simulink model "if_mode"  (R2022b)
settings: Solver=FixedStepAuto  StartTime=0.0  StopTime=10  FixedStep=1e-4  RelTol=1e-3
values from neighbouring files (symbols this model uses):
  CurrKi = 35.0    [if_mode.sldd]
  CurrKp = 0.17    [if_mode.sldd]
  flux = 0.016884    [if_mode.sldd]
  Pn = 4.0    [if_mode.sldd]
undefined symbols (not defined in the file or in its folder): curr_d_ki, curr_d_kp, curr_q_ki, curr_q_kp, DiscIntNeverNeededParam
libraries: slpidlib x4, mcbplantlib x1, autolibpmsmexterior x1
settings Model: DataDictionary=if_mode.sldd  Creator=SSC  LastModifiedBy=SSC
settings OptimizationCC: DefaultParameterBehavior=Inlined  UseDivisionForNetSlopeComputation=on  GainParamInheritBuiltInType=on  UseFloatMulNetSlope=on  InlineInvariantSignals=on  PassReuseOutputArgsAs=Individual arguments  ZeroExternalMemoryAtStartup=off  ZeroInternalMemoryAtStartup=off  NoFixptDivByZeroProtection=on  EfficientFloat2IntCast=on  LifeSpan=1  OptimizeBlockOrder=speed  DifferentSizesBufferReuse=on  EfficientTunableParamExpr=on
settings DebuggingCC: ParameterOverflowMsg=none  ParameterUnderflowMsg=error  ParameterTunabilityLossMsg=error
settings HardwareCC: ProdBitPerPointer=32  ProdBitPerSizeT=32  ProdBitPerPtrDiffT=32  ProdLargestAtomicInteger=Long  ProdLargestAtomicFloat=Double  ProdWordSize=32  ProdLongLongMode=on  ProdHWDeviceType=ARM Compatible->ARM Cortex-M
settings SFSimCC: MATLABDynamicMemAlloc=off
settings RTWCC: Description=Embedded Coder  SystemTargetFile=ert.tlc  TemplateMakefile=ert_default_tmf  GenerateReport=on  LaunchReport=on
settings CodeAppCC: ForceParamTrailComments=on  IgnoreCustomStorageClasses=off  OperatorAnnotations=on  SimulinkDataObjDesc=on  SFDataObjDesc=on  CustomSymbolStrGlobalVar=rt$N$M  CustomSymbolStrType=$N$M  CustomSymbolStrFcn=$N$M$F  CustomSymbolStrMacro=$N$M  InsertBlockDesc=on
settings ERTTargetCC: TargetLangStandard=C99 (ISO)  CodeReplacementLibrary=ARM Cortex-M  GenerateSampleERTMain=on  IncludeMdlTerminateFcn=off  CombineSignalStateStructs=on  SupportAbsoluteTime=off  SupportComplex=off  SupportNonInlinedSFcns=on  InlinedParameterPlacement=NonHierarchical  ERTCustomFileTemplate=example_file_process.tlc  ERTFilePackagingFormat=CompactWithDataFile

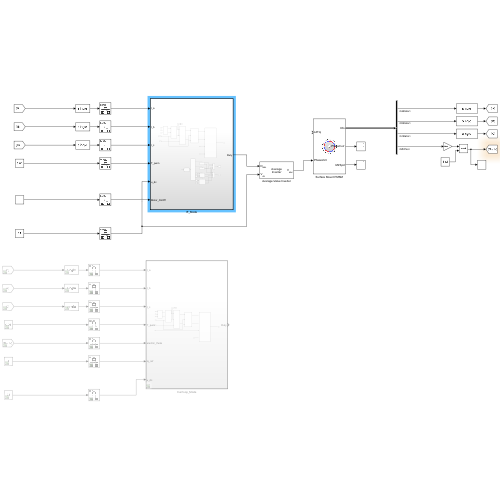
[thumbnail: Simulink's stored preview of the top-level diagram]
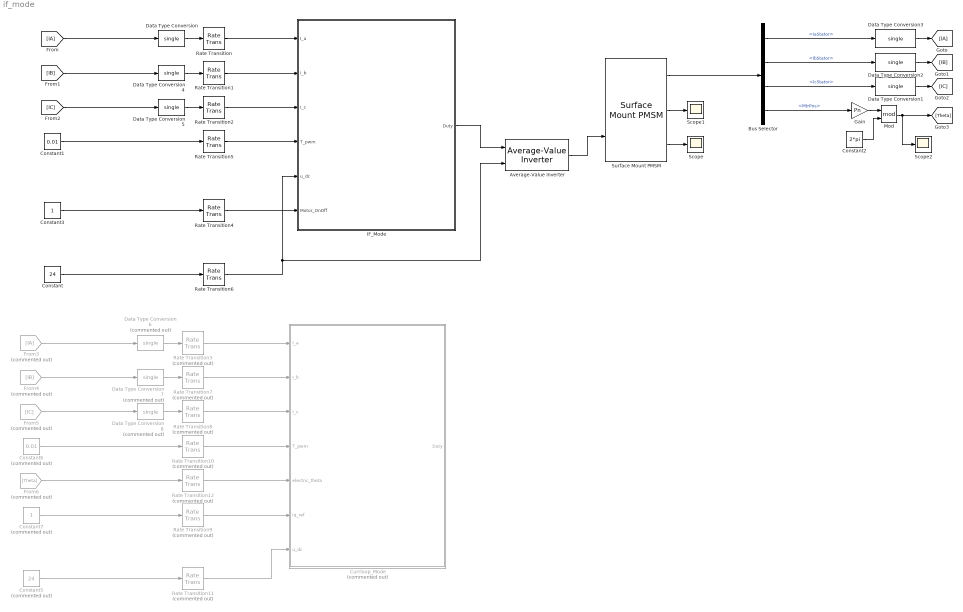
== system if_mode ==
  Average-Value Inverter : mcbplantlib/Average-Value Inverter
      settings: LibrarySourceBlock=mcblib/Electrical Systems/Inverters/Average-Value Inverter
  Bus Selector : BusSelector  OutputSignals=IaStator,IbStator,IcStator,MtrPos
  Constant : Constant  Value=24  OutDataTypeStr=single
  Constant1 : Constant  Value=0.01  OutDataTypeStr=single
  Constant2 : Constant  Value=2*pi  OutDataTypeStr=single
  Constant3 : Constant  OutDataTypeStr=single
  Constant5 : Constant  Commented=on  Value=24  OutDataTypeStr=single
  Constant6 : Constant  Commented=on  Value=0.01  OutDataTypeStr=single
  Constant7 : Constant  Commented=on  OutDataTypeStr=single
  Currloop_Mode : Subsystem  Commented=on  TreatAsAtomicUnit=on
  Data Type Conversion{,1..5} (6 alike) : DataTypeConversion  OutDataTypeStr=single  SaturateOnIntegerOverflow=off  RndMeth=Floor
  Data Type Conversion6 : DataTypeConversion  Commented=on  OutDataTypeStr=single  SaturateOnIntegerOverflow=off  RndMeth=Floor
  Data Type Conversion7 : DataTypeConversion  Commented=on  OutDataTypeStr=single  SaturateOnIntegerOverflow=off  RndMeth=Floor
  Data Type Conversion8 : DataTypeConversion  Commented=on  OutDataTypeStr=single  SaturateOnIntegerOverflow=off  RndMeth=Floor
  From3 : From  Commented=on  GotoTag=IA
  From4 : From  Commented=on  GotoTag=IB
  From5 : From  Commented=on  GotoTag=IC
  From6 : From  Commented=on  GotoTag=Theta
  Gain : Gain  Gain=Pn  OutDataTypeStr=single
  IF_Mode : Subsystem  TreatAsAtomicUnit=on
  Mod : Math  Operator=mod
  Rate Transition{,1..2,4..6} (6 alike) : RateTransition
  Rate Transition{3,7..12} (7 alike) : RateTransition  Commented=on
  Scope : Scope
  Scope1 : Scope
  Scope2 : Scope
  Surface Mount PMSM : autolibpmsmexterior/Surface Mount PMSM  port_config=Torque  sim_type=Discrete  Ts=1e-4  P=Pn  Rs=Rs  Ldq_=L  KConstText=Permanent flux linkage constant (lambda_pm):  lambda_pm=flux  Ke=223  Kt=1.323  mechanical=[75e-6,8e-5,0]  idq0=[0 0]  theta_init=0  omega_init=0  KConst=flux  lambda_pm_calc=flux  RefBlkName='autolibpmsmexterior/Surface Mount PMSM'  aMode=5  Ldq="[0.0017      0.0017]"
  wires:
  Constant/1 -> Rate Transition6/1
  Average-Value Inverter/1 -> Surface Mount PMSM/2
  Surface Mount PMSM/1 -> Bus Selector/1
  Bus Selector/1 -> Data Type Conversion3/1  "<IaStator>"
  Bus Selector/2 -> Data Type Conversion2/1  "<IbStator>"
  Bus Selector/3 -> Data Type Conversion1/1  "<IcStator>"
  Bus Selector/4 -> Gain/1  "<MtrPos>"
  Gain/1 -> Mod/1
  Mod/1 -> Scope2/1, [Theta]
  Data Type Conversion1/1 -> [IC]
  Data Type Conversion2/1 -> [IB]
  Data Type Conversion3/1 -> [IA]
  Surface Mount PMSM/3 -> Scope/1
  Surface Mount PMSM/2 -> Scope1/1
  Constant2/1 -> Mod/2
  Rate Transition2/1 -> IF_Mode/3(I_c)
  Rate Transition1/1 -> IF_Mode/2(I_b)
  Data Type Conversion/1 -> Rate Transition/1
  Data Type Conversion4/1 -> Rate Transition1/1
  [IA] -> Data Type Conversion/1
  Data Type Conversion5/1 -> Rate Transition2/1
  [IC] -> Data Type Conversion5/1
  [IB] -> Data Type Conversion4/1
  Rate Transition/1 -> IF_Mode/1(I_a)
  Rate Transition6/1 -> Average-Value Inverter/2, IF_Mode/5(u_dc)
  Constant1/1 -> Rate Transition5/1
  Rate Transition5/1 -> IF_Mode/4(T_pwm)
  Constant3/1 -> Rate Transition4/1
  Rate Transition4/1 -> IF_Mode/6(Motor_OnOff)
  Rate Transition3/1 -> Currloop_Mode/1(I_a)
  From4/1 -> Data Type Conversion7/1
  Data Type Conversion6/1 -> Rate Transition3/1
  From3/1 -> Data Type Conversion6/1
  From5/1 -> Data Type Conversion8/1
  Rate Transition11/1 -> Currloop_Mode/7(u_dc)
  Constant6/1 -> Rate Transition10/1
  Rate Transition8/1 -> Currloop_Mode/3(I_c)
  Constant5/1 -> Rate Transition11/1
  Data Type Conversion8/1 -> Rate Transition8/1
  Rate Transition7/1 -> Currloop_Mode/2(I_b)
  Constant7/1 -> Rate Transition9/1
  Data Type Conversion7/1 -> Rate Transition7/1
  Rate Transition9/1 -> Currloop_Mode/6(iq_ref)
  Rate Transition12/1 -> Currloop_Mode/5(electric_theta)
  From6/1 -> Rate Transition12/1
  Rate Transition10/1 -> Currloop_Mode/4(T_pwm)
  IF_Mode/1(Duty) -> Average-Value Inverter/1

== system if_mode/Currloop_Mode ==
  I_a : Inport
  I_b : Inport  Port=2
  I_c : Inport  Port=3
  T_pwm : Inport  Port=4
  electric_theta : Inport  Port=5
  iq_ref : Inport  Port=6
  u_dc : Inport  Port=7
  AntiPark : Subsystem
  Clark : Subsystem
  Curr_PI_Controller : Subsystem
  Park : Subsystem
  SVPWM : Subsystem
  Scope1 : Scope  NumInputPorts=2
  Duty : Outport
  wires:
  Clark/2(I_beta) -> Park/2(i_beta)  "i_beta"
  AntiPark/2(u_beta) -> SVPWM/2(U_beta)
  Park/2(i_q) -> Scope1/2, Curr_PI_Controller/2(iq_fdbk)  "i_q"
  I_c/1 -> Clark/3(I_c)
  Clark/1(I_alpha) -> Park/1(i_alpha)  "i_alpha"
  electric_theta/1 -> AntiPark/3(electric_theta), Park/3(electric_theta)
  Park/1(i_d) -> Scope1/1, Curr_PI_Controller/1(id_fdbk)  "i_d"
  Curr_PI_Controller/1(ud_ref) -> AntiPark/1(u_d)
  AntiPark/1(u_alpha) -> SVPWM/1(U_alpha)
  Curr_PI_Controller/2(uq_ref) -> AntiPark/2(u_q)
  I_a/1 -> Clark/1(I_a)
  SVPWM/1(Duty) -> Duty/1
  u_dc/1 -> SVPWM/4(u_dc)
  T_pwm/1 -> SVPWM/3(T_pwm)
  I_b/1 -> Clark/2(I_b)
  iq_ref/1 -> Curr_PI_Controller/3(iq_ref)

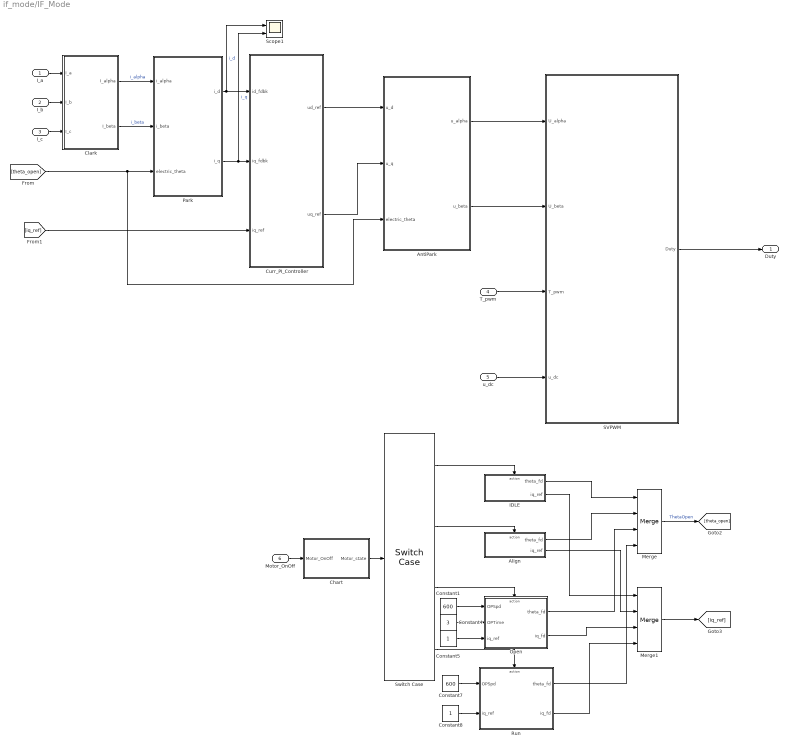
== system if_mode/IF_Mode ==
  I_a : Inport
  I_b : Inport  Port=2
  I_c : Inport  Port=3
  T_pwm : Inport  Port=4
  u_dc : Inport  Port=5
  Motor_OnOff : Inport  Port=6
  Align : Subsystem  TreatAsAtomicUnit=on
  AntiPark : Subsystem
  Chart : Stateflow chart  TreatAsAtomicUnit=on
  Clark : Subsystem
  Constant1 : Constant  Value=600  OutDataTypeStr=single
  Constant4 : Constant  Value=3  OutDataTypeStr=single
  Constant5 : Constant  OutDataTypeStr=single
  Constant7 : Constant  Value=600  OutDataTypeStr=single
  Constant8 : Constant  OutDataTypeStr=single
  Curr_PI_Controller : Subsystem
  IDLE : Subsystem  TreatAsAtomicUnit=on
  Merge : Merge  Inputs=4
  Merge1 : Merge  Inputs=4
  Open : Subsystem  TreatAsAtomicUnit=on
  Park : Subsystem
  Run : Subsystem  TreatAsAtomicUnit=on
  SVPWM : Subsystem
  Scope1 : Scope  NumInputPorts=2
  Switch Case : SwitchCase  CaseConditions={1,2,3,4}  ShowDefaultCase=off
  Duty : Outport
  wires:
  Clark/2(I_beta) -> Park/2(i_beta)  "i_beta"
  AntiPark/2(u_beta) -> SVPWM/2(U_beta)
  Park/2(i_q) -> Scope1/2, Curr_PI_Controller/2(iq_fdbk)  "i_q"
  I_c/1 -> Clark/3(I_c)
  Clark/1(I_alpha) -> Park/1(i_alpha)  "i_alpha"
  [theta_open] -> AntiPark/3(electric_theta), Park/3(electric_theta)
  Park/1(i_d) -> Scope1/1, Curr_PI_Controller/1(id_fdbk)  "i_d"
  Curr_PI_Controller/1(ud_ref) -> AntiPark/1(u_d)
  AntiPark/1(u_alpha) -> SVPWM/1(U_alpha)
  Curr_PI_Controller/2(uq_ref) -> AntiPark/2(u_q)
  I_a/1 -> Clark/1(I_a)
  SVPWM/1(Duty) -> Duty/1
  u_dc/1 -> SVPWM/4(u_dc)
  T_pwm/1 -> SVPWM/3(T_pwm)
  I_b/1 -> Clark/2(I_b)
  [iq_ref] -> Curr_PI_Controller/3(iq_ref)
  Switch Case/1 -> IDLE/Action
  Motor_OnOff/1 -> Chart/1(Motor_OnOff)
  Constant5/1 -> Open/3(iq_ref)
  Switch Case/2 -> Align/Action
  Constant4/1 -> Open/2(OPTime)
  Merge/1 -> [theta_open]  "ThetaOpen"
  Constant8/1 -> Run/2(iq_ref)
  Constant1/1 -> Open/1(OPSpd)
  Merge1/1 -> [iq_ref]
  Chart/1(Motor_state) -> Switch Case/1
  Constant7/1 -> Run/1(OPSpd)
  Switch Case/4 -> Run/Action
  Switch Case/3 -> Open/Action
  IDLE/1(theta_fd) -> Merge/1
  Align/1(theta_fd) -> Merge/2
  Open/1(theta_fd) -> Merge/3
  Run/1(theta_fd) -> Merge/4
  Run/2(iq_fd) -> Merge1/4
  Open/2(iq_fd) -> Merge1/3
  Align/2(iq_ref) -> Merge1/2
  IDLE/2(iq_ref) -> Merge1/1

== system if_mode/Currloop_Mode/AntiPark ==
  u_d : Inport
  u_q : Inport  Port=2
  electric_theta : Inport  Port=3
  Add : Sum  Inputs=+-
  Add1 : Sum
  Product{,1..3} (4 alike) : Product
  Scope : Scope  NumInputPorts=2
  Trigonometric Function : Trigonometry
  Trigonometric Function1 : Trigonometry  Operator=cos
  u_alpha : Outport
  u_beta : Outport  Port=2
  wires:
  electric_theta/1 -> Trigonometric Function1/1, Trigonometric Function/1
  u_d/1 -> Product2/1, Product/1
  Trigonometric Function1/1 -> Product/2, Product1/2
  u_q/1 -> Product1/1, Product3/1
  Trigonometric Function/1 -> Product2/2, Product3/2
  Product/1 -> Add/1
  Product3/1 -> Add/2
  Add/1 -> Scope/1, u_alpha/1
  Product2/1 -> Add1/1
  Product1/1 -> Add1/2
  Add1/1 -> Scope/2, u_beta/1

== system if_mode/Currloop_Mode/Clark ==
  I_a : Inport
  I_b : Inport  Port=2
  I_c : Inport  Port=3
  Add : Sum
  Add1 : Sum  Inputs=+-
  Add2 : Sum  Inputs=+-
  Gain : Gain  Gain=2/3
  Gain1 : Gain  Gain=1/3
  Gain2 : Gain  Gain=sqrt(3)/3
  I_alpha : Outport
  I_beta : Outport  Port=2
  wires:
  I_a/1 -> Gain/1
  I_b/1 -> Add1/1, Add/1
  I_c/1 -> Add/2, Add1/2
  Add/1 -> Gain1/1
  Add1/1 -> Gain2/1
  Gain/1 -> Add2/1
  Gain1/1 -> Add2/2
  Add2/1 -> I_alpha/1
  Gain2/1 -> I_beta/1

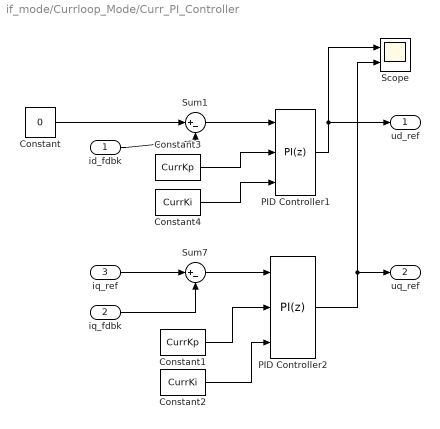
== system if_mode/Currloop_Mode/Curr_PI_Controller ==
  id_fdbk : Inport  OutDataTypeStr=single
  iq_fdbk : Inport  Port=2  OutDataTypeStr=single
  iq_ref : Inport  Port=3  OutDataTypeStr=single
  Constant : Constant  Value=0  OutDataTypeStr=single
  Constant1 : Constant  Value=CurrKp  OutDataTypeStr=single
  Constant2 : Constant  Value=CurrKi  OutDataTypeStr=single
  Constant3 : Constant  Value=CurrKp  OutDataTypeStr=single
  Constant4 : Constant  Value=CurrKi  OutDataTypeStr=single
  PID Controller1 : slpidlib/PID Controller  Controller=PI  Form=Parallel  TimeDomain=Discrete-time  UseExternalTs=off  SampleTime=-1  IntegratorMethod=Forward Euler  FilterMethod=Forward Euler  ControllerParametersSource=external  P=curr_d_kp  I=curr_d_ki  UseKiTs=off  D=0  N=100  UseFilter=on  TunerSelectOption=Transfer Function Based (PID Tuner App)  InitialConditionSource=internal  InitialConditionForIntegrator=0  InitialConditionForFilter=0  DifferentiatorICPrevScaledInput=0  ExternalReset=none  TrackingMode=off  Kt=1  LimitOutput=on  SatLimitsSource=internal  UpperSaturationLimit=24*0.9/sqrt(3)  LowerSaturationLimit=-24*0.9/sqrt(3)  LinearizeAsGain=on  AntiWindupMode=clamping  Kb=1  LimitIntegrator=off  UpperIntegratorSaturationLimit=inf  LowerIntegratorSaturationLimit=-inf  PGainOutDataTypeStr=single  PProdOutDataTypeStr=single  POutMin=[]  POutMax=[]  IGainOutDataTypeStr=int16  IProdOutDataTypeStr=int16  IOutMin=[]  IOutMax=[]  DOutMin=[]  DOutMax=[]  NOutMin=[]  NOutMax=[]  SumOutDataTypeStr=single  SumOutMin=[]  SumOutMax=[]  SaturationOutDataTypeStr=single  SaturationOutMin=[]  SaturationOutMax=[]  PParamMin=[]  PParamMax=[]  IParamMin=[]  IParamMax=[]  DParamMin=[]  DParamMax=[]  NParamMin=[]  NParamMax=[]  KbParamMin=[]  KbParamMax=[]  KtParamMin=[]  KtParamMax=[]  KbOutMin=[]  KbOutMax=[]  KtOutMin=[]  KtOutMax=[]  IntegratorOutMin=[]  IntegratorOutMax=[]  FilterOutMin=[]  FilterOutMax=[]  SumI1OutMin=[]  SumI1OutMax=[]  SumI2OutMin=[]  SumI2OutMax=[]  SumI3OutMin=[]  SumI3OutMax=[]  SumI4OutMin=[]  SumI4OutMax=[]  SumDOutMin=[]  SumDOutMax=[]  DifferentiatorOutMin=[]  DifferentiatorOutMax=[]  FilterDiffOutCoefMin=[]  FilterDiffOutCoefMax=[]  ReciprocalOutMin=[]  ReciprocalOutMax=[]  SumDenOutMin=[]  SumDenOutMax=[]  SumNumOutMin=[]  SumNumOutMax=[]  DivideOutMin=[]  DivideOutMax=[]  UdiffTsProdOutMin=[]  UdiffTsProdOutMax=[]  NTsProdOutMin=[]  NTsProdOutMax=[]  UintegralTsProdOutMin=[]  UintegralTsProdOutMax=[]  UngainTsProdOutMin=[]  UngainTsProdOutMax=[]  ClampingZeroOutDataTypeStr=Inherit: Inherit via back propagation  ClampingZeroOutMin=[]  ClampingZeroOutMax=[]  FilterDenConstantOutDataTypeStr=Inherit: Inherit via back propagation  FilterDenConstantOutMin=[]  FilterDenConstantOutMax=[]  PCopyOutDataTypeStr=Inherit: Inherit via back propagation  PCopyOutMin=[]  PCopyOutMax=[]  NCopyOutDataTypeStr=Inherit: Inherit via back propagation  NCopyOutMin=[]  NCopyOutMax=[]  IntegratorContinuousStateAttributes=''  IntegratorStateMustResolveToSignalObject=off  IntegratorRTWStateStorageClass=Auto  FilterContinuousStateAttributes=''  FilterStateMustResolveToSignalObject=off  FilterRTWStateStorageClass=Auto  ParallelPVariant=ExternalParameters  IdealPVariant=Disabled  IVariant=ExternalParameters  DVariant=Disabled  IntegratorVariant=Discrete  SatVariant=Enabled  AWVariant=DiscClampingParallel  PCopyVariant=Disabled  TRVariant=Disabled  FdbkBlocksVariant=Forward  IdealPFdbkVariant=Disabled  SatFdbkVariant=Disabled  DerivativeFilterVariant=Disabled  NVariant=Disabled  NCopyVariant=Disabled_SignalSpec  FilterICVariant=Disabled  IntegratorICVariant=InternalICs  ExternalResetVariant=Disabled  TRSumVariant=Passthrough  SumFdbkVariant=Disabled  SumVariant=Sum_PI  TsampFilterVariant=InternalTs  TsampNgainVariant=Passthrough  TsampIntegralVariant=Passthrough  ExternalSaturationOutDataTypeStr=Inherit: Same as second input
  PID Controller2 : slpidlib/PID Controller  Controller=PI  Form=Parallel  TimeDomain=Discrete-time  UseExternalTs=off  SampleTime=-1  IntegratorMethod=Forward Euler  FilterMethod=Forward Euler  ControllerParametersSource=external  P=curr_q_kp  I=curr_q_ki  UseKiTs=off  D=0  N=100  UseFilter=on  TunerSelectOption=Transfer Function Based (PID Tuner App)  InitialConditionSource=internal  InitialConditionForIntegrator=0  InitialConditionForFilter=0  DifferentiatorICPrevScaledInput=0  ExternalReset=none  TrackingMode=off  Kt=1  LimitOutput=on  SatLimitsSource=internal  UpperSaturationLimit=24*0.9/sqrt(3)  LowerSaturationLimit=-24*0.9/sqrt(3)  LinearizeAsGain=on  AntiWindupMode=clamping  Kb=1  LimitIntegrator=off  UpperIntegratorSaturationLimit=inf  LowerIntegratorSaturationLimit=-inf  PGainOutDataTypeStr=single  PProdOutDataTypeStr=single  POutMin=[]  POutMax=[]  IGainOutDataTypeStr=single  IProdOutDataTypeStr=single  IOutMin=[]  IOutMax=[]  DOutMin=[]  DOutMax=[]  NOutMin=[]  NOutMax=[]  SumOutDataTypeStr=single  SumOutMin=[]  SumOutMax=[]  SaturationOutDataTypeStr=single  SaturationOutMin=[]  SaturationOutMax=[]  PParamMin=[]  PParamMax=[]  IParamMin=[]  IParamMax=[]  DParamMin=[]  DParamMax=[]  NParamMin=[]  NParamMax=[]  KbParamMin=[]  KbParamMax=[]  KtParamMin=[]  KtParamMax=[]  KbOutMin=[]  KbOutMax=[]  KtOutMin=[]  KtOutMax=[]  IntegratorOutMin=[]  IntegratorOutMax=[]  FilterOutMin=[]  FilterOutMax=[]  SumI1OutMin=[]  SumI1OutMax=[]  SumI2OutMin=[]  SumI2OutMax=[]  SumI3OutMin=[]  SumI3OutMax=[]  SumI4OutMin=[]  SumI4OutMax=[]  SumDOutMin=[]  SumDOutMax=[]  DifferentiatorOutMin=[]  DifferentiatorOutMax=[]  FilterDiffOutCoefMin=[]  FilterDiffOutCoefMax=[]  ReciprocalOutMin=[]  ReciprocalOutMax=[]  SumDenOutMin=[]  SumDenOutMax=[]  SumNumOutMin=[]  SumNumOutMax=[]  DivideOutMin=[]  DivideOutMax=[]  UdiffTsProdOutMin=[]  UdiffTsProdOutMax=[]  NTsProdOutMin=[]  NTsProdOutMax=[]  UintegralTsProdOutMin=[]  UintegralTsProdOutMax=[]  UngainTsProdOutMin=[]  UngainTsProdOutMax=[]  ClampingZeroOutDataTypeStr=Inherit: Inherit via back propagation  ClampingZeroOutMin=[]  ClampingZeroOutMax=[]  FilterDenConstantOutDataTypeStr=Inherit: Inherit via back propagation  FilterDenConstantOutMin=[]  FilterDenConstantOutMax=[]  PCopyOutDataTypeStr=Inherit: Inherit via back propagation  PCopyOutMin=[]  PCopyOutMax=[]  NCopyOutDataTypeStr=Inherit: Inherit via back propagation  NCopyOutMin=[]  NCopyOutMax=[]  IntegratorContinuousStateAttributes=''  IntegratorStateMustResolveToSignalObject=off  IntegratorRTWStateStorageClass=Auto  FilterContinuousStateAttributes=''  FilterStateMustResolveToSignalObject=off  FilterRTWStateStorageClass=Auto  ParallelPVariant=ExternalParameters  IdealPVariant=Disabled  IVariant=ExternalParameters  DVariant=Disabled  IntegratorVariant=Discrete  SatVariant=Enabled  AWVariant=DiscClampingParallel  PCopyVariant=Disabled  TRVariant=Disabled  FdbkBlocksVariant=Forward  IdealPFdbkVariant=Disabled  SatFdbkVariant=Disabled  DerivativeFilterVariant=Disabled  NVariant=Disabled  NCopyVariant=Disabled_SignalSpec  FilterICVariant=Disabled  IntegratorICVariant=InternalICs  ExternalResetVariant=Disabled  TRSumVariant=Passthrough  SumFdbkVariant=Disabled  SumVariant=Sum_PI  TsampFilterVariant=InternalTs  TsampNgainVariant=Passthrough  TsampIntegralVariant=Passthrough  ExternalSaturationOutDataTypeStr=Inherit: Same as second input
  Scope : Scope  NumInputPorts=2
  Sum1 : Sum  Inputs=|+-  AccumDataTypeStr=single  OutDataTypeStr=single
  Sum7 : Sum  Inputs=|+-  AccumDataTypeStr=single  OutDataTypeStr=single
  ud_ref : Outport  OutDataTypeStr=single
  uq_ref : Outport  Port=2  OutDataTypeStr=single
  wires:
  id_fdbk/1 -> Sum1/2
  Constant/1 -> Sum1/1
  iq_fdbk/1 -> Sum7/2
  Sum1/1 -> PID Controller1/1
  PID Controller1/1 -> Scope/1, ud_ref/1
  PID Controller2/1 -> Scope/2, uq_ref/1
  iq_ref/1 -> Sum7/1
  Constant3/1 -> PID Controller1/2
  Constant4/1 -> PID Controller1/3
  Constant1/1 -> PID Controller2/2
  Constant2/1 -> PID Controller2/3
  Sum7/1 -> PID Controller2/1

== system if_mode/Currloop_Mode/Park ==
  i_alpha : Inport
  i_beta : Inport  Port=2
  electric_theta : Inport  Port=3
  Add : Sum
  Add1 : Sum  Inputs=-+
  Product{,1..3} (4 alike) : Product
  Scope : Scope  NumInputPorts=2
  Trigonometric Function : Trigonometry
  Trigonometric Function1 : Trigonometry  Operator=cos
  i_d : Outport
  i_q : Outport  Port=2
  wires:
  electric_theta/1 -> Trigonometric Function1/1, Trigonometric Function/1
  i_alpha/1 -> Product2/1, Product/1
  Trigonometric Function1/1 -> Product3/2, Product/2
  i_beta/1 -> Product3/1, Product1/1
  Trigonometric Function/1 -> Product2/2, Product1/2
  Product/1 -> Add/1
  Product1/1 -> Add/2
  Product2/1 -> Add1/1
  Product3/1 -> Add1/2
  Add/1 -> Scope/1, i_d/1
  Add1/1 -> Scope/2, i_q/1

== system if_mode/Currloop_Mode/SVPWM ==
  U_alpha : Inport
  U_beta : Inport  Port=2
  T_pwm : Inport  Port=3
  u_dc : Inport  Port=4
  Constant : Constant
  Duty_Caculator : Subsystem
  Gain : Gain  Gain=2
  Mux : Mux  Inputs=3
  Sector_Select : Subsystem
  Sum : Sum  Inputs=|-+
  T4_T6_Caculator : Subsystem
  X_Y_Z_Caculator : Subsystem
  Duty : Outport
  wires:
  U_alpha/1 -> X_Y_Z_Caculator/1(u_alpha), Sector_Select/1(u_alpha)
  U_beta/1 -> X_Y_Z_Caculator/2(u_beta), Sector_Select/2(u_beta)
  T_pwm/1 -> Duty_Caculator/4(T_pwm), T4_T6_Caculator/5(T_pwm), X_Y_Z_Caculator/3(T_pwm)
  u_dc/1 -> X_Y_Z_Caculator/4(U_dc)
  X_Y_Z_Caculator/1(X) -> T4_T6_Caculator/2(X)
  X_Y_Z_Caculator/2(Y) -> T4_T6_Caculator/3(Y)
  X_Y_Z_Caculator/3(Z) -> T4_T6_Caculator/4(Z)
  Sector_Select/1(N) -> T4_T6_Caculator/1(N), Duty_Caculator/1(N)
  T4_T6_Caculator/2(T6) -> Duty_Caculator/3(T6)
  T4_T6_Caculator/1(T4) -> Duty_Caculator/2(T4)
  Duty_Caculator/2(Dutyb) -> Mux/2
  Duty_Caculator/1(Dutya) -> Mux/1
  Duty_Caculator/3(Dutyc) -> Mux/3
  Sum/1 -> Duty/1
  Constant/1 -> Sum/2
  Mux/1 -> Gain/1
  Gain/1 -> Sum/1

== system if_mode/IF_Mode/Align ==
  Action Port : ActionPort  ActionPortLabel=case [ 2 ]:
  Constant : Constant  Value=0  OutDataTypeStr=single
  Constant1 : Constant  Value=2  OutDataTypeStr=single
  theta_fd : Outport
  iq_ref : Outport  Port=2
  wires:
  Constant1/1 -> iq_ref/1
  Constant/1 -> theta_fd/1

== system if_mode/IF_Mode/AntiPark ==
  u_d : Inport
  u_q : Inport  Port=2
  electric_theta : Inport  Port=3
  Add : Sum  Inputs=+-
  Add1 : Sum
  Product{,1..3} (4 alike) : Product
  Scope : Scope  NumInputPorts=2
  Trigonometric Function : Trigonometry
  Trigonometric Function1 : Trigonometry  Operator=cos
  u_alpha : Outport
  u_beta : Outport  Port=2
  wires:
  electric_theta/1 -> Trigonometric Function1/1, Trigonometric Function/1
  u_d/1 -> Product2/1, Product/1
  Trigonometric Function1/1 -> Product/2, Product1/2
  u_q/1 -> Product1/1, Product3/1
  Trigonometric Function/1 -> Product2/2, Product3/2
  Product/1 -> Add/1
  Product3/1 -> Add/2
  Add/1 -> Scope/1, u_alpha/1
  Product2/1 -> Add1/1
  Product1/1 -> Add1/2
  Add1/1 -> Scope/2, u_beta/1

== system if_mode/IF_Mode/Clark ==
  I_a : Inport
  I_b : Inport  Port=2
  I_c : Inport  Port=3
  Add : Sum
  Add1 : Sum  Inputs=+-
  Add2 : Sum  Inputs=+-
  Gain : Gain  Gain=2/3
  Gain1 : Gain  Gain=1/3
  Gain2 : Gain  Gain=sqrt(3)/3
  I_alpha : Outport
  I_beta : Outport  Port=2
  wires:
  I_a/1 -> Gain/1
  I_b/1 -> Add1/1, Add/1
  I_c/1 -> Add/2, Add1/2
  Add/1 -> Gain1/1
  Add1/1 -> Gain2/1
  Gain/1 -> Add2/1
  Gain1/1 -> Add2/2
  Add2/1 -> I_alpha/1
  Gain2/1 -> I_beta/1

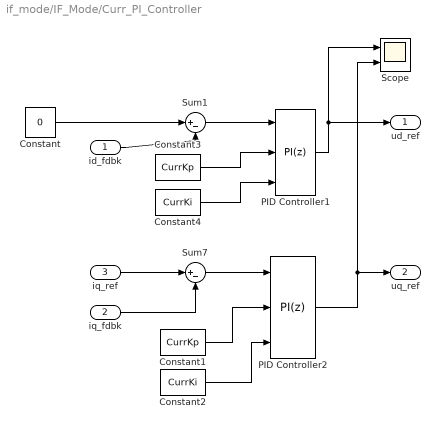
== system if_mode/IF_Mode/Curr_PI_Controller ==
  id_fdbk : Inport  OutDataTypeStr=single
  iq_fdbk : Inport  Port=2  OutDataTypeStr=single
  iq_ref : Inport  Port=3  OutDataTypeStr=single
  Constant : Constant  Value=0  OutDataTypeStr=single
  Constant1 : Constant  Value=CurrKp  OutDataTypeStr=single
  Constant2 : Constant  Value=CurrKi  OutDataTypeStr=single
  Constant3 : Constant  Value=CurrKp  OutDataTypeStr=single
  Constant4 : Constant  Value=CurrKi  OutDataTypeStr=single
  PID Controller1 : slpidlib/PID Controller  Controller=PI  Form=Parallel  TimeDomain=Discrete-time  UseExternalTs=off  SampleTime=-1  IntegratorMethod=Forward Euler  FilterMethod=Forward Euler  ControllerParametersSource=external  P=curr_d_kp  I=curr_d_ki  UseKiTs=off  D=0  N=100  UseFilter=on  TunerSelectOption=Transfer Function Based (PID Tuner App)  InitialConditionSource=internal  InitialConditionForIntegrator=0  InitialConditionForFilter=0  DifferentiatorICPrevScaledInput=0  ExternalReset=none  TrackingMode=off  Kt=1  LimitOutput=on  SatLimitsSource=internal  UpperSaturationLimit=24*0.9/sqrt(3)  LowerSaturationLimit=-24*0.9/sqrt(3)  LinearizeAsGain=on  AntiWindupMode=clamping  Kb=1  LimitIntegrator=off  UpperIntegratorSaturationLimit=inf  LowerIntegratorSaturationLimit=-inf  PGainOutDataTypeStr=single  PProdOutDataTypeStr=single  POutMin=[]  POutMax=[]  IGainOutDataTypeStr=int16  IProdOutDataTypeStr=int16  IOutMin=[]  IOutMax=[]  DOutMin=[]  DOutMax=[]  NOutMin=[]  NOutMax=[]  SumOutDataTypeStr=single  SumOutMin=[]  SumOutMax=[]  SaturationOutDataTypeStr=single  SaturationOutMin=[]  SaturationOutMax=[]  PParamMin=[]  PParamMax=[]  IParamMin=[]  IParamMax=[]  DParamMin=[]  DParamMax=[]  NParamMin=[]  NParamMax=[]  KbParamMin=[]  KbParamMax=[]  KtParamMin=[]  KtParamMax=[]  KbOutMin=[]  KbOutMax=[]  KtOutMin=[]  KtOutMax=[]  IntegratorOutMin=[]  IntegratorOutMax=[]  FilterOutMin=[]  FilterOutMax=[]  SumI1OutMin=[]  SumI1OutMax=[]  SumI2OutMin=[]  SumI2OutMax=[]  SumI3OutMin=[]  SumI3OutMax=[]  SumI4OutMin=[]  SumI4OutMax=[]  SumDOutMin=[]  SumDOutMax=[]  DifferentiatorOutMin=[]  DifferentiatorOutMax=[]  FilterDiffOutCoefMin=[]  FilterDiffOutCoefMax=[]  ReciprocalOutMin=[]  ReciprocalOutMax=[]  SumDenOutMin=[]  SumDenOutMax=[]  SumNumOutMin=[]  SumNumOutMax=[]  DivideOutMin=[]  DivideOutMax=[]  UdiffTsProdOutMin=[]  UdiffTsProdOutMax=[]  NTsProdOutMin=[]  NTsProdOutMax=[]  UintegralTsProdOutMin=[]  UintegralTsProdOutMax=[]  UngainTsProdOutMin=[]  UngainTsProdOutMax=[]  ClampingZeroOutDataTypeStr=Inherit: Inherit via back propagation  ClampingZeroOutMin=[]  ClampingZeroOutMax=[]  FilterDenConstantOutDataTypeStr=Inherit: Inherit via back propagation  FilterDenConstantOutMin=[]  FilterDenConstantOutMax=[]  PCopyOutDataTypeStr=Inherit: Inherit via back propagation  PCopyOutMin=[]  PCopyOutMax=[]  NCopyOutDataTypeStr=Inherit: Inherit via back propagation  NCopyOutMin=[]  NCopyOutMax=[]  IntegratorContinuousStateAttributes=''  IntegratorStateMustResolveToSignalObject=off  IntegratorRTWStateStorageClass=Auto  FilterContinuousStateAttributes=''  FilterStateMustResolveToSignalObject=off  FilterRTWStateStorageClass=Auto  ParallelPVariant=ExternalParameters  IdealPVariant=Disabled  IVariant=ExternalParameters  DVariant=Disabled  IntegratorVariant=Discrete  SatVariant=Enabled  AWVariant=DiscClampingParallel  PCopyVariant=Disabled  TRVariant=Disabled  FdbkBlocksVariant=Forward  IdealPFdbkVariant=Disabled  SatFdbkVariant=Disabled  DerivativeFilterVariant=Disabled  NVariant=Disabled  NCopyVariant=Disabled_SignalSpec  FilterICVariant=Disabled  IntegratorICVariant=InternalICs  ExternalResetVariant=Disabled  TRSumVariant=Passthrough  SumFdbkVariant=Disabled  SumVariant=Sum_PI  TsampFilterVariant=InternalTs  TsampNgainVariant=Passthrough  TsampIntegralVariant=Passthrough  ExternalSaturationOutDataTypeStr=Inherit: Same as second input
  PID Controller2 : slpidlib/PID Controller  Controller=PI  Form=Parallel  TimeDomain=Discrete-time  UseExternalTs=off  SampleTime=-1  IntegratorMethod=Forward Euler  FilterMethod=Forward Euler  ControllerParametersSource=external  P=curr_q_kp  I=curr_q_ki  UseKiTs=off  D=0  N=100  UseFilter=on  TunerSelectOption=Transfer Function Based (PID Tuner App)  InitialConditionSource=internal  InitialConditionForIntegrator=0  InitialConditionForFilter=0  DifferentiatorICPrevScaledInput=0  ExternalReset=none  TrackingMode=off  Kt=1  LimitOutput=on  SatLimitsSource=internal  UpperSaturationLimit=24*0.9/sqrt(3)  LowerSaturationLimit=-24*0.9/sqrt(3)  LinearizeAsGain=on  AntiWindupMode=clamping  Kb=1  LimitIntegrator=off  UpperIntegratorSaturationLimit=inf  LowerIntegratorSaturationLimit=-inf  PGainOutDataTypeStr=single  PProdOutDataTypeStr=single  POutMin=[]  POutMax=[]  IGainOutDataTypeStr=single  IProdOutDataTypeStr=single  IOutMin=[]  IOutMax=[]  DOutMin=[]  DOutMax=[]  NOutMin=[]  NOutMax=[]  SumOutDataTypeStr=single  SumOutMin=[]  SumOutMax=[]  SaturationOutDataTypeStr=single  SaturationOutMin=[]  SaturationOutMax=[]  PParamMin=[]  PParamMax=[]  IParamMin=[]  IParamMax=[]  DParamMin=[]  DParamMax=[]  NParamMin=[]  NParamMax=[]  KbParamMin=[]  KbParamMax=[]  KtParamMin=[]  KtParamMax=[]  KbOutMin=[]  KbOutMax=[]  KtOutMin=[]  KtOutMax=[]  IntegratorOutMin=[]  IntegratorOutMax=[]  FilterOutMin=[]  FilterOutMax=[]  SumI1OutMin=[]  SumI1OutMax=[]  SumI2OutMin=[]  SumI2OutMax=[]  SumI3OutMin=[]  SumI3OutMax=[]  SumI4OutMin=[]  SumI4OutMax=[]  SumDOutMin=[]  SumDOutMax=[]  DifferentiatorOutMin=[]  DifferentiatorOutMax=[]  FilterDiffOutCoefMin=[]  FilterDiffOutCoefMax=[]  ReciprocalOutMin=[]  ReciprocalOutMax=[]  SumDenOutMin=[]  SumDenOutMax=[]  SumNumOutMin=[]  SumNumOutMax=[]  DivideOutMin=[]  DivideOutMax=[]  UdiffTsProdOutMin=[]  UdiffTsProdOutMax=[]  NTsProdOutMin=[]  NTsProdOutMax=[]  UintegralTsProdOutMin=[]  UintegralTsProdOutMax=[]  UngainTsProdOutMin=[]  UngainTsProdOutMax=[]  ClampingZeroOutDataTypeStr=Inherit: Inherit via back propagation  ClampingZeroOutMin=[]  ClampingZeroOutMax=[]  FilterDenConstantOutDataTypeStr=Inherit: Inherit via back propagation  FilterDenConstantOutMin=[]  FilterDenConstantOutMax=[]  PCopyOutDataTypeStr=Inherit: Inherit via back propagation  PCopyOutMin=[]  PCopyOutMax=[]  NCopyOutDataTypeStr=Inherit: Inherit via back propagation  NCopyOutMin=[]  NCopyOutMax=[]  IntegratorContinuousStateAttributes=''  IntegratorStateMustResolveToSignalObject=off  IntegratorRTWStateStorageClass=Auto  FilterContinuousStateAttributes=''  FilterStateMustResolveToSignalObject=off  FilterRTWStateStorageClass=Auto  ParallelPVariant=ExternalParameters  IdealPVariant=Disabled  IVariant=ExternalParameters  DVariant=Disabled  IntegratorVariant=Discrete  SatVariant=Enabled  AWVariant=DiscClampingParallel  PCopyVariant=Disabled  TRVariant=Disabled  FdbkBlocksVariant=Forward  IdealPFdbkVariant=Disabled  SatFdbkVariant=Disabled  DerivativeFilterVariant=Disabled  NVariant=Disabled  NCopyVariant=Disabled_SignalSpec  FilterICVariant=Disabled  IntegratorICVariant=InternalICs  ExternalResetVariant=Disabled  TRSumVariant=Passthrough  SumFdbkVariant=Disabled  SumVariant=Sum_PI  TsampFilterVariant=InternalTs  TsampNgainVariant=Passthrough  TsampIntegralVariant=Passthrough  ExternalSaturationOutDataTypeStr=Inherit: Same as second input
  Scope : Scope  NumInputPorts=2
  Sum1 : Sum  Inputs=|+-  AccumDataTypeStr=single  OutDataTypeStr=single
  Sum7 : Sum  Inputs=|+-  AccumDataTypeStr=single  OutDataTypeStr=single
  ud_ref : Outport  OutDataTypeStr=single
  uq_ref : Outport  Port=2  OutDataTypeStr=single
  wires:
  id_fdbk/1 -> Sum1/2
  Constant/1 -> Sum1/1
  iq_fdbk/1 -> Sum7/2
  Sum1/1 -> PID Controller1/1
  PID Controller1/1 -> Scope/1, ud_ref/1
  PID Controller2/1 -> Scope/2, uq_ref/1
  iq_ref/1 -> Sum7/1
  Constant3/1 -> PID Controller1/2
  Constant4/1 -> PID Controller1/3
  Constant1/1 -> PID Controller2/2
  Constant2/1 -> PID Controller2/3
  Sum7/1 -> PID Controller2/1

== system if_mode/IF_Mode/IDLE ==
  Action Port : ActionPort  ActionPortLabel=case [ 1 ]:
  Constant : Constant  Value=0  OutDataTypeStr=single
  Constant1 : Constant  Value=0  OutDataTypeStr=single
  theta_fd : Outport
  iq_ref : Outport  Port=2
  wires:
  Constant1/1 -> iq_ref/1
  Constant/1 -> theta_fd/1

== system if_mode/IF_Mode/Open ==
  OPSpd : Inport  OutDataTypeStr=single  PortDimensions=1
  OPTime : Inport  Port=2  OutDataTypeStr=single  PortDimensions=1
  iq_ref : Inport  Port=3
  Action Port : ActionPort  ActionPortLabel=case [ 3 ]:
  Constant1 : Constant  Value=2*pi  OutDataTypeStr=single
  Constant4 : Constant  OutDataTypeStr=single
  Discrete-Time Integrator : DiscreteIntegrator  SampleTime=-1  ICPrevOutput=DiscIntNeverNeededParam  ICPrevScaledInput=DiscIntNeverNeededParam
  Discrete-Time Integrator1 : DiscreteIntegrator  SampleTime=-1  ICPrevOutput=DiscIntNeverNeededParam  ICPrevScaledInput=DiscIntNeverNeededParam
  Divide : Product  Inputs=*/  OutDataTypeStr=single
  Gain : Gain  Gain=Pn
  Gain1 : Gain  Gain=pi/30  OutDataTypeStr=single
  Mod : Math  Operator=mod
  Product : Product  OutDataTypeStr=single
  theta_fd : Outport
  iq_fd : Outport  Port=2
  wires:
  iq_ref/1 -> iq_fd/1
  Constant4/1 -> Divide/1
  Constant1/1 -> Mod/2
  Discrete-Time Integrator1/1 -> Mod/1
  Gain1/1 -> Gain/1
  Divide/1 -> Product/2
  Discrete-Time Integrator/1 -> Discrete-Time Integrator1/1
  Mod/1 -> theta_fd/1
  Gain/1 -> Product/1
  Product/1 -> Discrete-Time Integrator/1
  OPSpd/1 -> Gain1/1
  OPTime/1 -> Divide/2

== system if_mode/IF_Mode/Park ==
  i_alpha : Inport
  i_beta : Inport  Port=2
  electric_theta : Inport  Port=3
  Add : Sum
  Add1 : Sum  Inputs=-+
  Product{,1..3} (4 alike) : Product
  Scope : Scope  NumInputPorts=2
  Trigonometric Function : Trigonometry
  Trigonometric Function1 : Trigonometry  Operator=cos
  i_d : Outport
  i_q : Outport  Port=2
  wires:
  electric_theta/1 -> Trigonometric Function1/1, Trigonometric Function/1
  i_alpha/1 -> Product2/1, Product/1
  Trigonometric Function1/1 -> Product3/2, Product/2
  i_beta/1 -> Product3/1, Product1/1
  Trigonometric Function/1 -> Product2/2, Product1/2
  Product/1 -> Add/1
  Product1/1 -> Add/2
  Product2/1 -> Add1/1
  Product3/1 -> Add1/2
  Add/1 -> Scope/1, i_d/1
  Add1/1 -> Scope/2, i_q/1

== system if_mode/IF_Mode/Run ==
  OPSpd : Inport  OutDataTypeStr=single  PortDimensions=1
  iq_ref : Inport  Port=2
  Action Port : ActionPort  ActionPortLabel=case [ 4 ]:
  Constant1 : Constant  Value=2*pi  OutDataTypeStr=single
  Discrete-Time Integrator1 : DiscreteIntegrator  SampleTime=-1  ICPrevOutput=DiscIntNeverNeededParam  ICPrevScaledInput=DiscIntNeverNeededParam
  Gain : Gain  Gain=Pn
  Gain1 : Gain  Gain=pi/30  OutDataTypeStr=single
  Mod : Math  Operator=mod
  theta_fd : Outport
  iq_fd : Outport  Port=2
  wires:
  iq_ref/1 -> iq_fd/1
  OPSpd/1 -> Gain1/1
  Discrete-Time Integrator1/1 -> Mod/1
  Constant1/1 -> Mod/2
  Gain/1 -> Discrete-Time Integrator1/1
  Gain1/1 -> Gain/1
  Mod/1 -> theta_fd/1

== system if_mode/IF_Mode/SVPWM ==
  U_alpha : Inport
  U_beta : Inport  Port=2
  T_pwm : Inport  Port=3
  u_dc : Inport  Port=4
  Constant : Constant
  Duty_Caculator : Subsystem
  Gain : Gain  Gain=2
  Mux : Mux  Inputs=3
  Sector_Select : Subsystem
  Sum : Sum  Inputs=|-+
  T4_T6_Caculator : Subsystem
  X_Y_Z_Caculator : Subsystem
  Duty : Outport
  wires:
  U_alpha/1 -> X_Y_Z_Caculator/1(u_alpha), Sector_Select/1(u_alpha)
  U_beta/1 -> X_Y_Z_Caculator/2(u_beta), Sector_Select/2(u_beta)
  T_pwm/1 -> Duty_Caculator/4(T_pwm), T4_T6_Caculator/5(T_pwm), X_Y_Z_Caculator/3(T_pwm)
  u_dc/1 -> X_Y_Z_Caculator/4(U_dc)
  X_Y_Z_Caculator/1(X) -> T4_T6_Caculator/2(X)
  X_Y_Z_Caculator/2(Y) -> T4_T6_Caculator/3(Y)
  X_Y_Z_Caculator/3(Z) -> T4_T6_Caculator/4(Z)
  Sector_Select/1(N) -> T4_T6_Caculator/1(N), Duty_Caculator/1(N)
  T4_T6_Caculator/2(T6) -> Duty_Caculator/3(T6)
  T4_T6_Caculator/1(T4) -> Duty_Caculator/2(T4)
  Duty_Caculator/2(Dutyb) -> Mux/2
  Duty_Caculator/1(Dutya) -> Mux/1
  Duty_Caculator/3(Dutyc) -> Mux/3
  Sum/1 -> Duty/1
  Constant/1 -> Sum/2
  Mux/1 -> Gain/1
  Gain/1 -> Sum/1

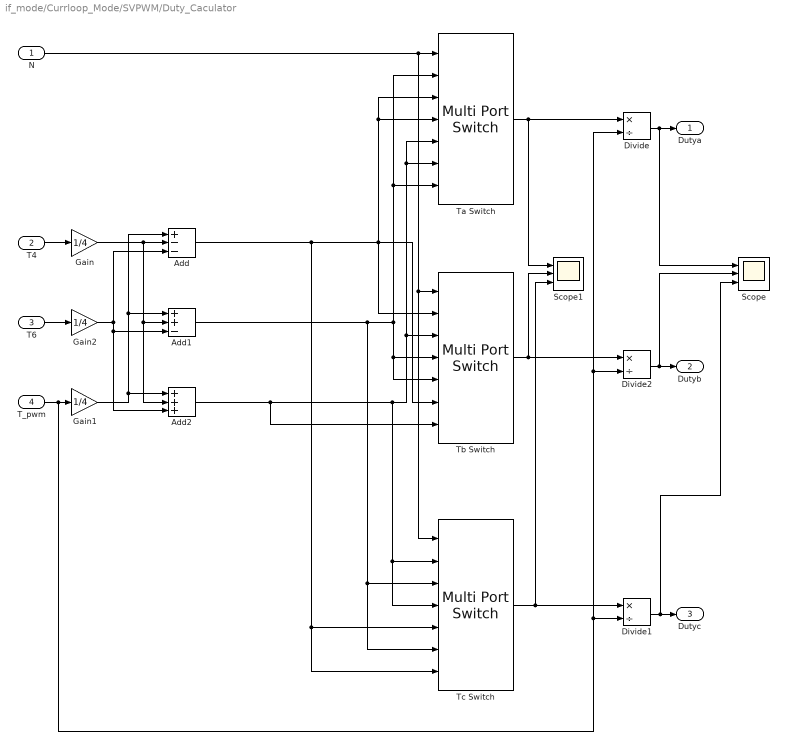
== system if_mode/Currloop_Mode/SVPWM/Duty_Caculator ==
  N : Inport
  T4 : Inport  Port=2
  T6 : Inport  Port=3
  T_pwm : Inport  Port=4
  Add : Sum  Inputs=+--
  Add1 : Sum  Inputs=++-
  Add2 : Sum  Inputs=+++
  Divide : Product  Inputs=*/
  Divide1 : Product  Inputs=*/
  Divide2 : Product  Inputs=*/
  Gain : Gain  Gain=1/4
  Gain1 : Gain  Gain=1/4
  Gain2 : Gain  Gain=1/4
  Scope : Scope  NumInputPorts=3
  Scope1 : Scope  NumInputPorts=3
  Ta Switch : MultiPortSwitch  Inputs=6  SaturateOnIntegerOverflow=off  InputSameDT=off
  Tb Switch : MultiPortSwitch  Inputs=6  SaturateOnIntegerOverflow=off  InputSameDT=off
  Tc Switch : MultiPortSwitch  Inputs=6  SaturateOnIntegerOverflow=off  InputSameDT=off
  Dutya : Outport
  Dutyb : Outport  Port=2
  Dutyc : Outport  Port=3
  wires:
  T4/1 -> Gain/1
  T6/1 -> Gain2/1
  T_pwm/1 -> Divide2/2, Divide/2, Divide1/2, Gain1/1
  Gain1/1 -> Add2/1, Add1/1, Add/1
  Gain/1 -> Add2/2, Add1/2, Add/2
  Gain2/1 -> Add2/3, Add1/3, Add/3
  N/1 -> Tc Switch/1, Tb Switch/1, Ta Switch/1
  Add/1 -> Tc Switch/7, Tc Switch/5, Tb Switch/6, Ta Switch/3, Ta Switch/4, Tb Switch/2
  Add1/1 -> Tc Switch/3, Tc Switch/6, Ta Switch/7, Ta Switch/2, Tb Switch/5, Tb Switch/4
  Add2/1 -> Tb Switch/7, Ta Switch/5, Ta Switch/6, Tb Switch/3, Tc Switch/4, Tc Switch/2
  Ta Switch/1 -> Scope1/1, Divide/1
  Tb Switch/1 -> Scope1/2, Divide2/1
  Tc Switch/1 -> Scope1/3, Divide1/1
  Divide/1 -> Scope/1, Dutya/1
  Divide1/1 -> Scope/3, Dutyc/1
  Divide2/1 -> Scope/2, Dutyb/1

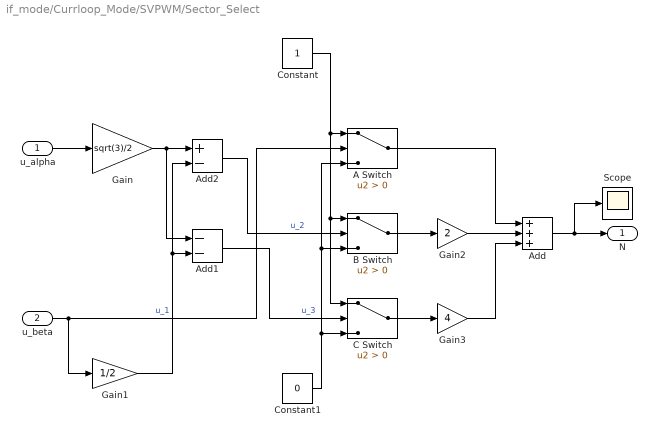
== system if_mode/Currloop_Mode/SVPWM/Sector_Select ==
  u_alpha : Inport
  u_beta : Inport  Port=2
  " A Switch" : Switch  Criteria=u2 > Threshold  SaturateOnIntegerOverflow=off  InputSameDT=off
  " B Switch" : Switch  Criteria=u2 > Threshold  SaturateOnIntegerOverflow=off  InputSameDT=off
  " C Switch" : Switch  Criteria=u2 > Threshold  SaturateOnIntegerOverflow=off  InputSameDT=off
  Add : Sum  Inputs=+++
  Add1 : Sum  Inputs=--
  Add2 : Sum  Inputs=+-
  Constant : Constant
  Constant1 : Constant  Value=0
  Gain : Gain  Gain=sqrt(3)/2
  Gain1 : Gain  Gain=1/2
  Gain2 : Gain  Gain=2
  Gain3 : Gain  Gain=4
  Scope : Scope
  N : Outport
  wires:
  Constant/1 -> " C Switch"/1, " B Switch"/1, " A Switch"/1
  Constant1/1 -> " C Switch"/3, " B Switch"/3, " A Switch"/3
  " A Switch"/1 -> Add/1
  Add/1 -> Scope/1, N/1
  " C Switch"/1 -> Gain3/1
  " B Switch"/1 -> Gain2/1
  u_beta/1 -> Gain1/1, " A Switch"/2  "u_1"
  u_alpha/1 -> Gain/1
  Gain/1 -> Add1/1, Add2/1
  Gain1/1 -> Add1/2, Add2/2
  Add2/1 -> " B Switch"/2  "u_2"
  Add1/1 -> " C Switch"/2  "u_3"
  Gain2/1 -> Add/2
  Gain3/1 -> Add/3

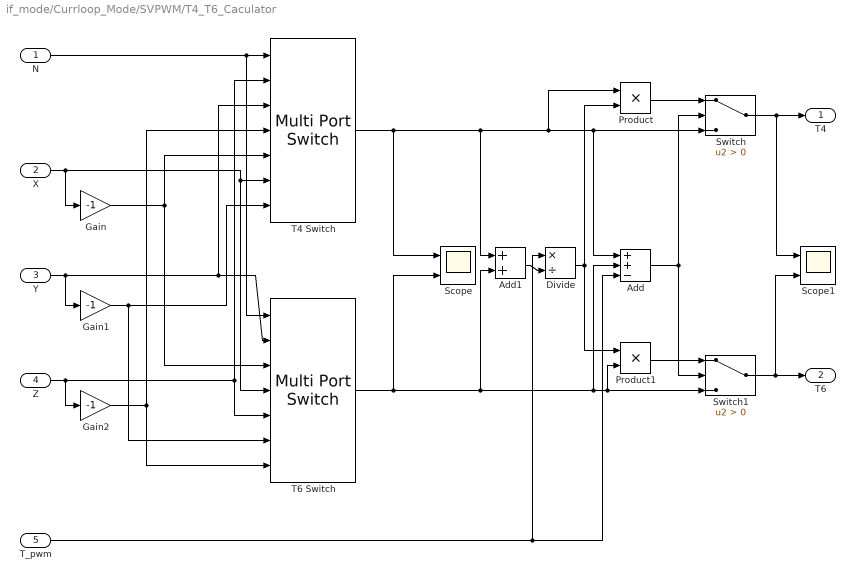
== system if_mode/Currloop_Mode/SVPWM/T4_T6_Caculator ==
  N : Inport
  X : Inport  Port=2
  Y : Inport  Port=3
  Z : Inport  Port=4
  T_pwm : Inport  Port=5
  Add : Sum  Inputs=++-
  Add1 : Sum
  Divide : Product  Inputs=*/
  Gain : Gain  Gain=-1
  Gain1 : Gain  Gain=-1
  Gain2 : Gain  Gain=-1
  Product : Product
  Product1 : Product
  Scope : Scope  NumInputPorts=2
  Scope1 : Scope  NumInputPorts=2
  Switch : Switch  Criteria=u2 > Threshold  SaturateOnIntegerOverflow=off  InputSameDT=off
  Switch1 : Switch  Criteria=u2 > Threshold  SaturateOnIntegerOverflow=off  InputSameDT=off
  T4 Switch : MultiPortSwitch  Inputs=6  SaturateOnIntegerOverflow=off  InputSameDT=off
  T6 Switch : MultiPortSwitch  Inputs=6  SaturateOnIntegerOverflow=off  InputSameDT=off
  T4 : Outport
  T6 : Outport  Port=2
  wires:
  Z/1 -> T4 Switch/2, T6 Switch/5, Gain2/1
  Y/1 -> Gain1/1, T4 Switch/3, T6 Switch/2
  X/1 -> T4 Switch/6, T6 Switch/4, Gain/1
  N/1 -> T6 Switch/1, T4 Switch/1
  Gain/1 -> T6 Switch/3, T4 Switch/5
  Gain2/1 -> T6 Switch/7, T4 Switch/4
  Gain1/1 -> T4 Switch/7, T6 Switch/6
  T4 Switch/1 -> Add1/1, Product/1, Add/1, Switch/3, Scope/1
  T6 Switch/1 -> Add1/2, Add/2, Switch1/3, Product1/2, Scope/2
  T_pwm/1 -> Add/3, Divide/1
  Add/1 -> Switch1/2, Switch/2
  Add1/1 -> Divide/2
  Product1/1 -> Switch1/1
  Product/1 -> Switch/1
  Divide/1 -> Product/2, Product1/1
  Switch/1 -> Scope1/1, T4/1
  Switch1/1 -> Scope1/2, T6/1

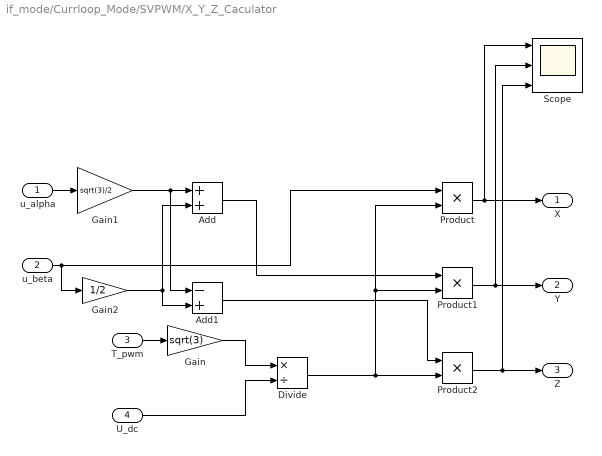
== system if_mode/Currloop_Mode/SVPWM/X_Y_Z_Caculator ==
  u_alpha : Inport
  u_beta : Inport  Port=2
  T_pwm : Inport  Port=3
  U_dc : Inport  Port=4
  Add : Sum
  Add1 : Sum  Inputs=-+
  Divide : Product  Inputs=*/
  Gain : Gain  Gain=sqrt(3)
  Gain1 : Gain  Gain=sqrt(3)/2
  Gain2 : Gain  Gain=1/2
  Product : Product
  Product1 : Product
  Product2 : Product
  Scope : Scope  NumInputPorts=3
  X : Outport
  Y : Outport  Port=2
  Z : Outport  Port=3
  wires:
  T_pwm/1 -> Gain/1
  U_dc/1 -> Divide/2
  Gain/1 -> Divide/1
  u_beta/1 -> Gain2/1, Product/1
  Divide/1 -> Product2/2, Product1/2, Product/2
  Product/1 -> Scope/1, X/1
  u_alpha/1 -> Gain1/1
  Gain1/1 -> Add1/1, Add/1
  Gain2/1 -> Add1/2, Add/2
  Add/1 -> Product1/1
  Product1/1 -> Scope/2, Y/1
  Add1/1 -> Product2/1
  Product2/1 -> Scope/3, Z/1

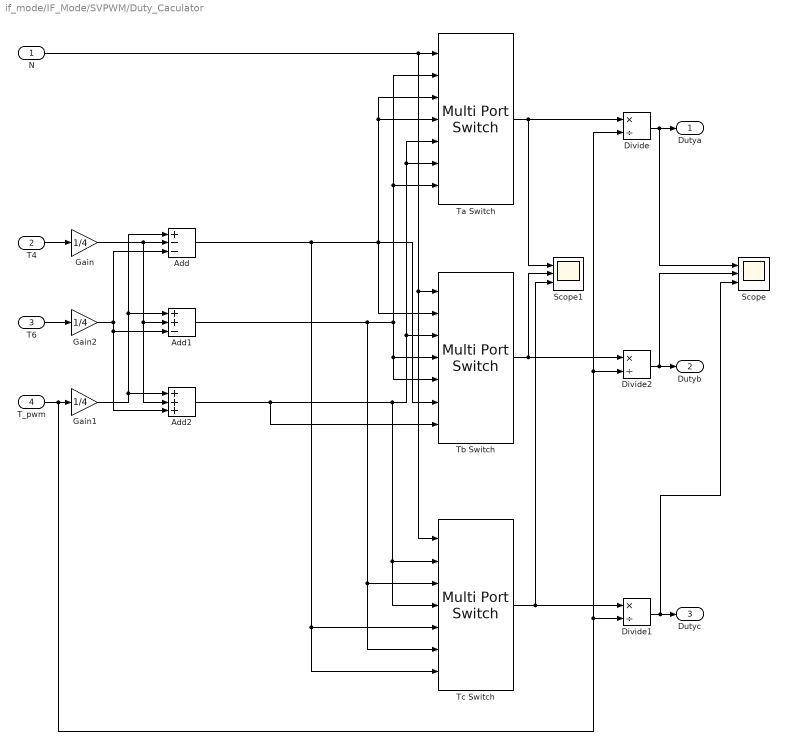
== system if_mode/IF_Mode/SVPWM/Duty_Caculator ==
  N : Inport
  T4 : Inport  Port=2
  T6 : Inport  Port=3
  T_pwm : Inport  Port=4
  Add : Sum  Inputs=+--
  Add1 : Sum  Inputs=++-
  Add2 : Sum  Inputs=+++
  Divide : Product  Inputs=*/
  Divide1 : Product  Inputs=*/
  Divide2 : Product  Inputs=*/
  Gain : Gain  Gain=1/4
  Gain1 : Gain  Gain=1/4
  Gain2 : Gain  Gain=1/4
  Scope : Scope  NumInputPorts=3
  Scope1 : Scope  NumInputPorts=3
  Ta Switch : MultiPortSwitch  Inputs=6  DiagnosticForDefault=None  SaturateOnIntegerOverflow=off  InputSameDT=off
  Tb Switch : MultiPortSwitch  Inputs=6  DiagnosticForDefault=None  SaturateOnIntegerOverflow=off  InputSameDT=off
  Tc Switch : MultiPortSwitch  Inputs=6  DiagnosticForDefault=None  SaturateOnIntegerOverflow=off  InputSameDT=off
  Dutya : Outport
  Dutyb : Outport  Port=2
  Dutyc : Outport  Port=3
  wires:
  T4/1 -> Gain/1
  T6/1 -> Gain2/1
  T_pwm/1 -> Divide2/2, Divide/2, Divide1/2, Gain1/1
  Gain1/1 -> Add2/1, Add1/1, Add/1
  Gain/1 -> Add2/2, Add1/2, Add/2
  Gain2/1 -> Add2/3, Add1/3, Add/3
  N/1 -> Tc Switch/1, Tb Switch/1, Ta Switch/1
  Add/1 -> Tc Switch/7, Tc Switch/5, Tb Switch/6, Ta Switch/3, Ta Switch/4, Tb Switch/2
  Add1/1 -> Tc Switch/3, Tc Switch/6, Ta Switch/7, Ta Switch/2, Tb Switch/5, Tb Switch/4
  Add2/1 -> Tb Switch/7, Ta Switch/5, Ta Switch/6, Tb Switch/3, Tc Switch/4, Tc Switch/2
  Ta Switch/1 -> Scope1/1, Divide/1
  Tb Switch/1 -> Scope1/2, Divide2/1
  Tc Switch/1 -> Scope1/3, Divide1/1
  Divide/1 -> Scope/1, Dutya/1
  Divide1/1 -> Scope/3, Dutyc/1
  Divide2/1 -> Scope/2, Dutyb/1

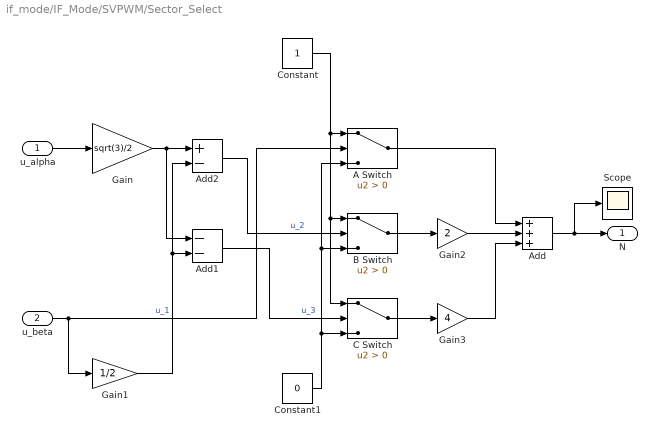
== system if_mode/IF_Mode/SVPWM/Sector_Select ==
  u_alpha : Inport
  u_beta : Inport  Port=2
  " A Switch" : Switch  Criteria=u2 > Threshold  SaturateOnIntegerOverflow=off  InputSameDT=off
  " B Switch" : Switch  Criteria=u2 > Threshold  SaturateOnIntegerOverflow=off  InputSameDT=off
  " C Switch" : Switch  Criteria=u2 > Threshold  SaturateOnIntegerOverflow=off  InputSameDT=off
  Add : Sum  Inputs=+++
  Add1 : Sum  Inputs=--
  Add2 : Sum  Inputs=+-
  Constant : Constant
  Constant1 : Constant  Value=0
  Gain : Gain  Gain=sqrt(3)/2
  Gain1 : Gain  Gain=1/2
  Gain2 : Gain  Gain=2
  Gain3 : Gain  Gain=4
  Scope : Scope
  N : Outport
  wires:
  Constant/1 -> " C Switch"/1, " B Switch"/1, " A Switch"/1
  Constant1/1 -> " C Switch"/3, " B Switch"/3, " A Switch"/3
  " A Switch"/1 -> Add/1
  Add/1 -> Scope/1, N/1
  " C Switch"/1 -> Gain3/1
  " B Switch"/1 -> Gain2/1
  u_beta/1 -> Gain1/1, " A Switch"/2  "u_1"
  u_alpha/1 -> Gain/1
  Gain/1 -> Add1/1, Add2/1
  Gain1/1 -> Add1/2, Add2/2
  Add2/1 -> " B Switch"/2  "u_2"
  Add1/1 -> " C Switch"/2  "u_3"
  Gain2/1 -> Add/2
  Gain3/1 -> Add/3

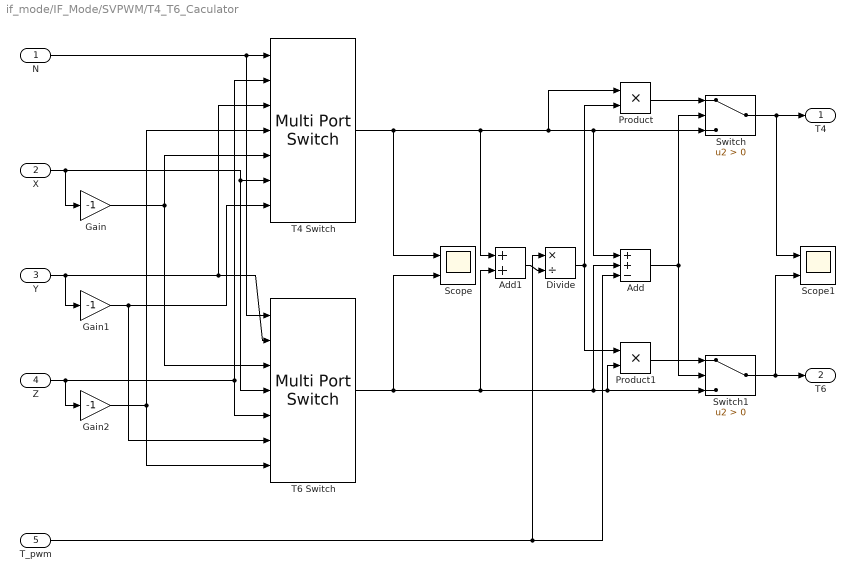
== system if_mode/IF_Mode/SVPWM/T4_T6_Caculator ==
  N : Inport
  X : Inport  Port=2
  Y : Inport  Port=3
  Z : Inport  Port=4
  T_pwm : Inport  Port=5
  Add : Sum  Inputs=++-
  Add1 : Sum
  Divide : Product  Inputs=*/
  Gain : Gain  Gain=-1
  Gain1 : Gain  Gain=-1
  Gain2 : Gain  Gain=-1
  Product : Product
  Product1 : Product
  Scope : Scope  NumInputPorts=2
  Scope1 : Scope  NumInputPorts=2
  Switch : Switch  Criteria=u2 > Threshold  SaturateOnIntegerOverflow=off  InputSameDT=off
  Switch1 : Switch  Criteria=u2 > Threshold  SaturateOnIntegerOverflow=off  InputSameDT=off
  T4 Switch : MultiPortSwitch  Inputs=6  DiagnosticForDefault=None  SaturateOnIntegerOverflow=off  InputSameDT=off
  T6 Switch : MultiPortSwitch  Inputs=6  DiagnosticForDefault=None  SaturateOnIntegerOverflow=off  InputSameDT=off
  T4 : Outport
  T6 : Outport  Port=2
  wires:
  Z/1 -> T4 Switch/2, T6 Switch/5, Gain2/1
  Y/1 -> Gain1/1, T4 Switch/3, T6 Switch/2
  X/1 -> T4 Switch/6, T6 Switch/4, Gain/1
  N/1 -> T6 Switch/1, T4 Switch/1
  Gain/1 -> T6 Switch/3, T4 Switch/5
  Gain2/1 -> T6 Switch/7, T4 Switch/4
  Gain1/1 -> T4 Switch/7, T6 Switch/6
  T4 Switch/1 -> Add1/1, Product/1, Add/1, Switch/3, Scope/1
  T6 Switch/1 -> Add1/2, Add/2, Switch1/3, Product1/2, Scope/2
  T_pwm/1 -> Add/3, Divide/1
  Add/1 -> Switch1/2, Switch/2
  Add1/1 -> Divide/2
  Product1/1 -> Switch1/1
  Product/1 -> Switch/1
  Divide/1 -> Product/2, Product1/1
  Switch/1 -> Scope1/1, T4/1
  Switch1/1 -> Scope1/2, T6/1

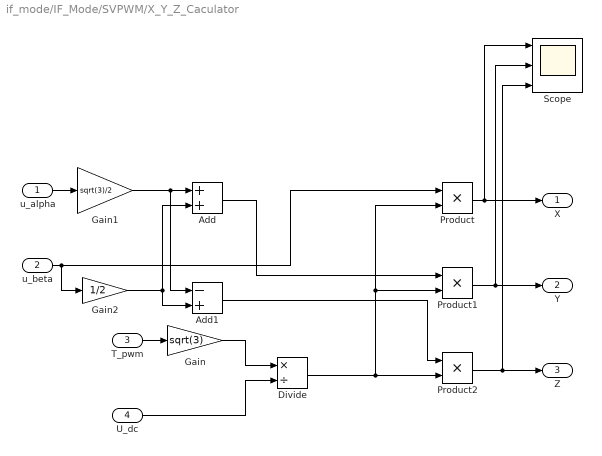
== system if_mode/IF_Mode/SVPWM/X_Y_Z_Caculator ==
  u_alpha : Inport
  u_beta : Inport  Port=2
  T_pwm : Inport  Port=3
  U_dc : Inport  Port=4
  Add : Sum
  Add1 : Sum  Inputs=-+
  Divide : Product  Inputs=*/
  Gain : Gain  Gain=sqrt(3)
  Gain1 : Gain  Gain=sqrt(3)/2
  Gain2 : Gain  Gain=1/2
  Product : Product
  Product1 : Product
  Product2 : Product
  Scope : Scope  NumInputPorts=3
  X : Outport
  Y : Outport  Port=2
  Z : Outport  Port=3
  wires:
  T_pwm/1 -> Gain/1
  U_dc/1 -> Divide/2
  Gain/1 -> Divide/1
  u_beta/1 -> Gain2/1, Product/1
  Divide/1 -> Product2/2, Product1/2, Product/2
  Product/1 -> Scope/1, X/1
  u_alpha/1 -> Gain1/1
  Gain1/1 -> Add1/1, Add/1
  Gain2/1 -> Add1/2, Add/2
  Add/1 -> Product1/1
  Product1/1 -> Scope/2, Y/1
  Add1/1 -> Product2/1
  Product2/1 -> Scope/3, Z/1

== stateflow chart if_mode/IF_Mode/Chart ==
  state RunStage
    en:
    du:
    Motor_state = 4;
  state OpenStage
    en:
    du:
    Motor_state = 3;
  state AlignStage
    en:
    du:
    Motor_state = 2;
  state IDLE
    en:
    du:
    Motor_state = 1;
  (default) -> IDLE
  IDLE -> AlignStage : [Motor_OnOff ==1]
  AlignStage -> OpenStage [order 1] : [after(1000,tick)]
  OpenStage -> RunStage [order 2] : [after(30000,tick) ]
  AlignStage -> IDLE [order 2] : [Motor_OnOff == 0]
  OpenStage -> IDLE [order 1] : [Motor_OnOff ==0]
  RunStage -> IDLE : [Motor_OnOff ==0]
  data: Motor_OnOff input; Motor_state output
